simulink model "W08_2_dock"  (R2024b)
settings: Solver=ode4  StartTime=0.0  StopTime=900  FixedStep=Ts_ctrl  RelTol=1e-3
InitFcn:
  | if ~exist('W08_dock_init','file'), addpath(fileparts(get_param('W08_2_dock','FileName'))); end, W08_dock_init('W08_2_dock')
StopFcn:
  | W08_dock_done('W08_2_dock')
values from neighbouring files (symbols this model uses):
  alloc_prm = [half_beam; l_bow; F_max; F_bow_max]    [W08_dock_setup.m]
  animate = 1    [W08_dock_setup.m]    (also in W08_setup.m)
  bow_on = 1    [W08_dock_setup.m]
  Delta = 10    [W08_dock_setup.m]    (also in W08_setup.m)
  dock_q = [dock_north; dock_east; dock_deg*pi/180; L_app; berth_side; R_dock; R_stop]    [W08_dock_setup.m]
  F_bow_max = 250    [W08_dock_setup.m]
  F_max = 500    [W08_dock_setup.m]    (also in W08_setup.m)
  half_beam = 1.027135    [W08_dock_setup.m]    (also in W08_setup.m)
  Izz = 653    [W08_dock_setup.m]    (also in W08_setup.m; build_w08_dock.m = p(2); build_w08_models.m = p(2))
  k_prop = 1000 * 0.004422 * 0.2^4    (= 0.0070752)    [W08_dock_setup.m]    (also in W08_setup.m)
  Kb = Ki_u / Kp_u    (= 0.333333333333)    [W08_dock_setup.m]
  Kd_psi = 200    [W08_dock_setup.m]    (also in W08_setup.m)
  Ki_u = 100    [W08_dock_setup.m]    (also in W08_setup.m)
  Ki_v = 100    [W08_dock_setup.m]
  Kp_psi = 400    [W08_dock_setup.m]    (also in W08_setup.m)
  Kp_u = 300    [W08_dock_setup.m]    (also in W08_setup.m)
  Kp_v = 300    [W08_dock_setup.m]
  Kp_x = 0.4    [W08_dock_setup.m]
  Kp_y = 0.4    [W08_dock_setup.m]
  l_bow = 0.75    [W08_dock_setup.m]
  loiter_radius = 18    [W08_dock_setup.m]    (also in W08_setup.m)
  loiter_turns = 1    [W08_dock_setup.m]    (also in W08_setup.m)
  loiter_wp = 3    [W08_dock_setup.m]    (also in W08_setup.m)
  loiter_xc = wp_north(loiter_wp)    [W08_dock_setup.m]    (also in W08_setup.m)
  loiter_yc = wp_east(loiter_wp)    [W08_dock_setup.m]    (also in W08_setup.m)
  m_usv = 211    [W08_dock_setup.m]    (also in W08_setup.m)
  n_bow_max = sqrt(F_bow_max / k_prop)    [W08_dock_setup.m]
  n_max = sqrt(F_max / k_prop)    [W08_dock_setup.m]    (also in W08_setup.m)
  Nr = 800    [W08_dock_setup.m]    (also in W08_setup.m)
  Nrr = 800    [W08_dock_setup.m]    (also in W08_setup.m; build_w08_dock.m = p(8); build_w08_models.m = p(8))
  p_c = 0.313    [W08_dock_setup.m]    (also in W08_setup.m)
  R_LOS = 5    [W08_dock_setup.m]    (also in W08_setup.m)
  tau_n = 0.30    (= 0.3)    [W08_dock_setup.m]    (also in W08_setup.m)
  Ts_ctrl = 0.05    [W08_dock_setup.m]    (also in W08_setup.m)
  u_max = 1.5    [W08_dock_setup.m]
  u_ref = 1.5    [W08_dock_setup.m]    (also in W08_setup.m)
  v_max = 0.6    [W08_dock_setup.m]
  wp_east = [  20   20   55   90   90 ]    [W08_dock_setup.m]    (also in W08_setup.m)
  wp_north = [ -20   50   20   50   10 ]    [W08_dock_setup.m]    (also in W08_setup.m)
  x0 = [0.1; 0; 0; 0; 0; psi_init]    [W08_dock_setup.m]    (also in W08_setup.m; W08_vrx_run.m = x0old;   x0(6) = psi0;   assignin('base','x0', x0); tidy_layout.m = min(P(:,1)))
  Xu = 100    [W08_dock_setup.m]    (also in W08_setup.m; build_w08_dock.m = p(3); build_w08_models.m = p(3))
  Xuu = 150    [W08_dock_setup.m]    (also in W08_setup.m; build_w08_dock.m = p(4); build_w08_models.m = p(4))
  Yv = 100    [W08_dock_setup.m]    (also in W08_setup.m; build_w08_dock.m = p(5); build_w08_models.m = p(5))
  Yvv = 100    [W08_dock_setup.m]    (also in W08_setup.m; build_w08_dock.m = p(6);'                newline  'Nr=p(7); build_w08_models.m = p(6);'                newline  'Nr=p(7))
libraries: slpidlib x2
settings Model: Creator=admin  LastModifiedBy=admin

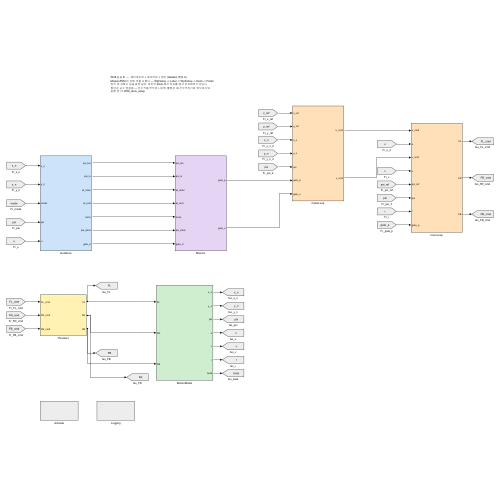
[thumbnail: Simulink's stored preview of the top-level diagram]
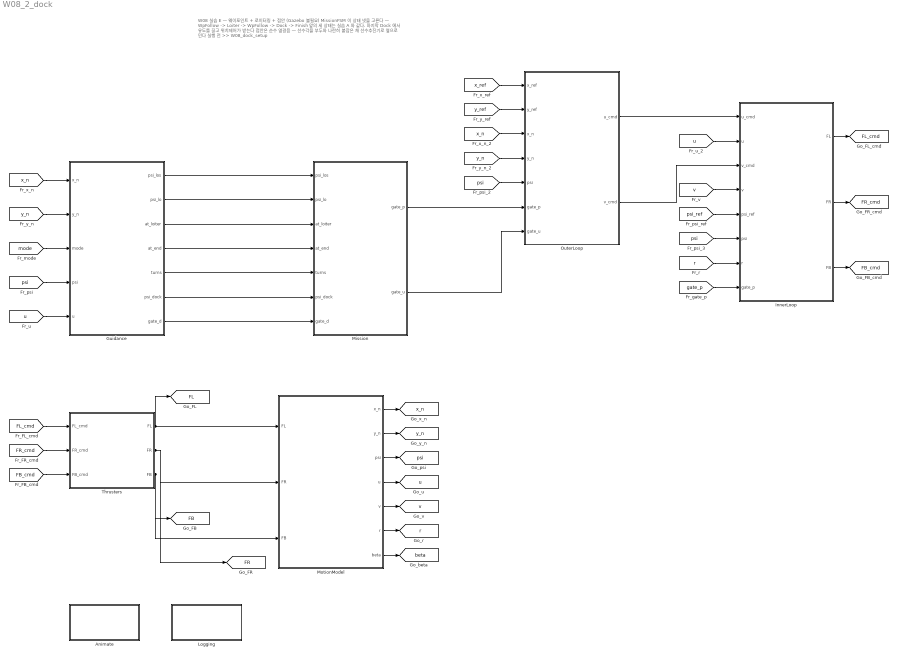
== system W08_2_dock ==
  note: W08 실습 E  —  웨이포인트 + 로이터링 + 접안 (Gazebo 불필요)
      | MissionFSM 이 상태 넷을 고른다 — WpFollow -> Loiter -> WpFollow -> Dock -> Finish
      | 앞의 세 상태는 실습 A 와 같다. 마지막 Dock 에서 유도를 끊고 위치제어가 받는다
      | 접안은 순수 옆걸음 — 선수각을 부두와 나란히 붙잡은 채 선수추진기로 옆으로 민다
      | 실행 전 >> W08_dock_setup
  Animate : Subsystem
  Guidance : Subsystem
  InnerLoop : Subsystem
  Logging : Subsystem
  Mission : Subsystem
  MotionModel : Subsystem
  OuterLoop : Subsystem
  Thrusters : Subsystem
  tag scope: FB=global, FB_cmd=global, FL=global, FL_cmd=global, FR=global, FR_cmd=global, beta=global, psi=global, r=global, u=global, v=global, x_n=global, y_n=global
  wires:
  OuterLoop/2(v_cmd) -> InnerLoop/3(v_cmd)
  OuterLoop/1(u_cmd) -> InnerLoop/1(u_cmd)
  Mission/1(gate_p) -> OuterLoop/6(gate_p)
  Guidance/7(gate_d) -> Mission/7(gate_d)
  Guidance/6(psi_dock) -> Mission/6(psi_dock)
  Guidance/5(turns) -> Mission/5(turns)
  Guidance/4(at_end) -> Mission/4(at_end)
  Guidance/3(at_loiter) -> Mission/3(at_loiter)
  Guidance/2(psi_lo) -> Mission/2(psi_lo)
  Guidance/1(psi_los) -> Mission/1(psi_los)
  Thrusters/2(FR) -> [FR], MotionModel/2(FR)
  Thrusters/1(FL) -> MotionModel/1(FL), [FL]
  Mission/2(gate_u) -> OuterLoop/7(gate_u)
  InnerLoop/1(FL) -> [FL_cmd]
  InnerLoop/2(FR) -> [FR_cmd]
  MotionModel/3(psi) -> [psi]
  MotionModel/4(u) -> [u]
  MotionModel/5(v) -> [v]
  MotionModel/1(x_n) -> [x_n]
  MotionModel/2(y_n) -> [y_n]
  [FL_cmd] -> Thrusters/1(FL_cmd)
  [FR_cmd] -> Thrusters/2(FR_cmd)
  [gate_p] -> InnerLoop/8(gate_p)
  [psi] -> InnerLoop/6(psi)
  [psi_ref] -> InnerLoop/5(psi_ref)
  [r] -> InnerLoop/7(r)
  [u] -> Guidance/5(u)
  [u] -> InnerLoop/2(u)
  [v] -> InnerLoop/4(v)
  [x_ref] -> OuterLoop/1(x_ref)
  [y_ref] -> OuterLoop/2(y_ref)
  InnerLoop/3(FB) -> [FB_cmd]
  MotionModel/7(beta) -> [beta]
  MotionModel/6(r) -> [r]
  [FB_cmd] -> Thrusters/3(FB_cmd)
  [psi] -> Guidance/4(psi)
  [x_n] -> OuterLoop/3(x_n)
  [y_n] -> OuterLoop/4(y_n)
  [mode] -> Guidance/3(mode)
  [psi] -> OuterLoop/5(psi)
  [y_n] -> Guidance/2(y_n)
  [x_n] -> Guidance/1(x_n)
  Thrusters/3(FB) -> [FB], MotionModel/3(FB)

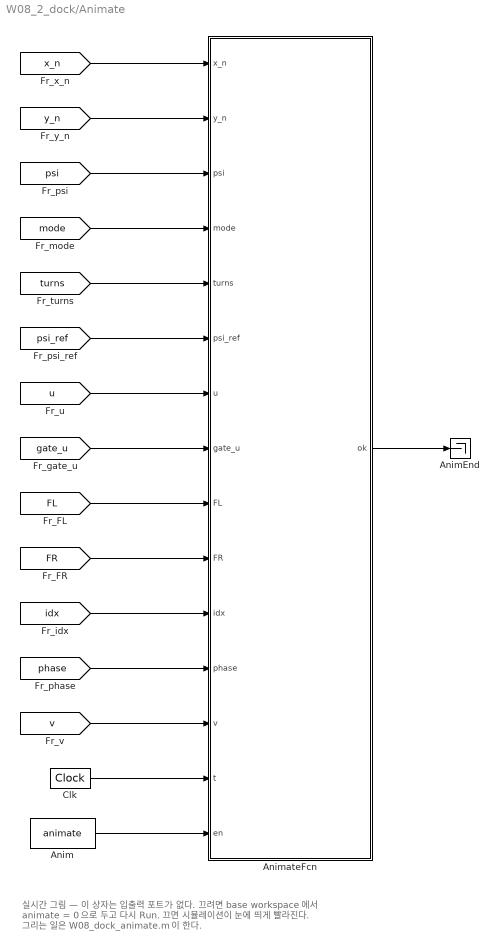
== system W08_2_dock/Animate ==
  note: 실시간 그림 — 이 상자는 입출력 포트가 없다.
      | 끄려면 base workspace 에서  animate = 0  으로 두고 다시 Run.
      | 끄면 시뮬레이션이 눈에 띄게 빨라진다.
      | 그리는 일은 W08_dock_animate.m 이 한다.
  Anim : Constant  Value=animate
  AnimEnd : Terminator
  AnimateFcn : MATLAB Function  TreatAsAtomicUnit=on
  Clk : DigitalClock  SampleTime=Ts_ctrl
  wires:
  [x_n] -> AnimateFcn/1(x_n)
  [y_n] -> AnimateFcn/2(y_n)
  [psi] -> AnimateFcn/3(psi)
  [mode] -> AnimateFcn/4(mode)
  [turns] -> AnimateFcn/5(turns)
  [psi_ref] -> AnimateFcn/6(psi_ref)
  [u] -> AnimateFcn/7(u)
  [gate_u] -> AnimateFcn/8(gate_u)
  [FL] -> AnimateFcn/9(FL)
  [FR] -> AnimateFcn/10(FR)
  [idx] -> AnimateFcn/11(idx)
  [phase] -> AnimateFcn/12(phase)
  [v] -> AnimateFcn/13(v)
  Clk/1 -> AnimateFcn/14(t)
  Anim/1 -> AnimateFcn/15(en)
  AnimateFcn/1(ok) -> AnimEnd/1

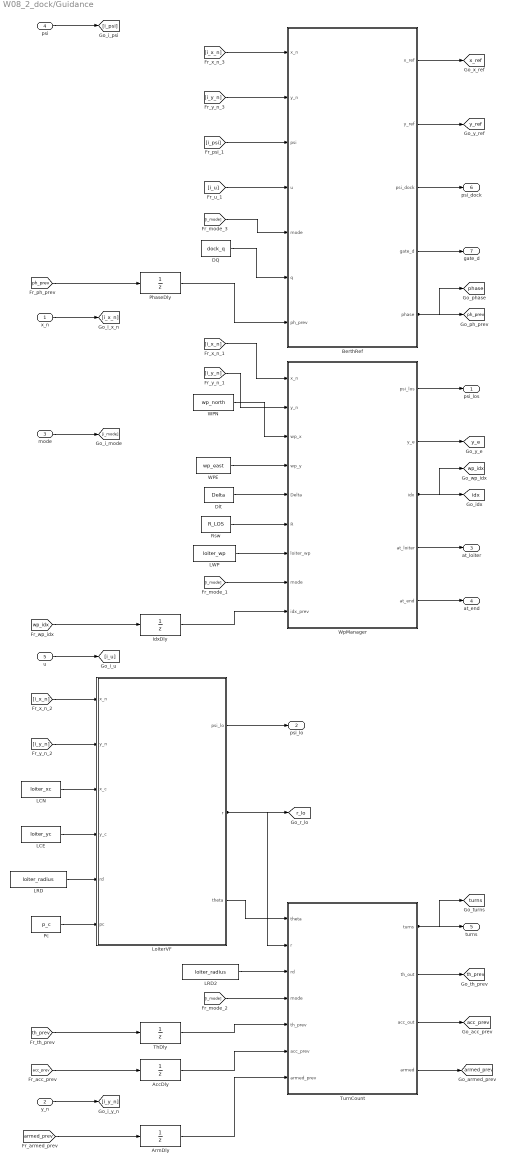
== system W08_2_dock/Guidance ==
  x_n : Inport
  y_n : Inport  Port=2
  mode : Inport  Port=3
  psi : Inport  Port=4
  u : Inport  Port=5
  AccDly : UnitDelay  Description=바퀴 수 계수기 — 표본 사이의 각 변화를 모아 감으므로 바로 앞 표본이 있어야 한다. 또한 TurnCount 가 낸 값이 TurnCount 로 되돌아와 대수 루프가 된다.  SampleTime=Ts_ctrl  HasFrameUpgradeWarning=on
  ArmDly : UnitDelay  Description=바퀴 수 계수기 — 표본 사이의 각 변화를 모아 감으므로 바로 앞 표본이 있어야 한다. 또한 TurnCount 가 낸 값이 TurnCount 로 되돌아와 대수 루프가 된다.  SampleTime=Ts_ctrl  HasFrameUpgradeWarning=on
  BerthRef : MATLAB Function  TreatAsAtomicUnit=on
  DQ : Constant  Value=dock_q
  Dlt : Constant  Value=Delta
  IdxDly : UnitDelay  Description=대수 루프 차단 + 사건 계수기 — 웨이포인트 번호는 정수이고, 유도부가 낸 값이 유도부로 되돌아온다. 미분방정식의 상태가 아니다.  InitialCondition=1  SampleTime=Ts_ctrl  HasFrameUpgradeWarning=on
  LCE : Constant  Value=loiter_yc
  LCN : Constant  Value=loiter_xc
  LRD : Constant  Value=loiter_radius
  LRD2 : Constant  Value=loiter_radius
  LWP : Constant  Value=loiter_wp
  LoiterVF : MATLAB Function  TreatAsAtomicUnit=on
  Pc : Constant  Value=p_c
  PhaseDly : UnitDelay  Description=대수 루프 차단 + 단계 걸쇠 — 접안 단계는 정수이고, 한 번 올라간 단계는 내려오지 않는다. 미분방정식의 상태가 아니다.  SampleTime=Ts_ctrl  HasFrameUpgradeWarning=on
  Rsw : Constant  Value=R_LOS
  ThDly : UnitDelay  Description=바퀴 수 계수기 — 표본 사이의 각 변화를 모아 감으므로 바로 앞 표본이 있어야 한다. 또한 TurnCount 가 낸 값이 TurnCount 로 되돌아와 대수 루프가 된다.  SampleTime=Ts_ctrl  HasFrameUpgradeWarning=on
  TurnCount : MATLAB Function  TreatAsAtomicUnit=on
  WPE : Constant  Value=wp_east
  WPN : Constant  Value=wp_north
  WpManager : MATLAB Function  TreatAsAtomicUnit=on
  psi_los : Outport
  psi_lo : Outport  Port=2
  at_loiter : Outport  Port=3
  at_end : Outport  Port=4
  turns : Outport  Port=5
  psi_dock : Outport  Port=6
  gate_d : Outport  Port=7
  tag scope: acc_prev=global, armed_prev=global, idx=global, ph_prev=global, phase=global, r_lo=global, th_prev=global, turns=global, wp_idx=global, x_ref=global, y_e=global, y_ref=global
  wires:
  WpManager/4(at_loiter) -> at_loiter/1
  psi/1 -> [i_psi]
  mode/1 -> [i_mode]
  LCE/1 -> LoiterVF/4(y_c)
  [ph_prev] -> PhaseDly/1
  LRD/1 -> LoiterVF/5(rd)
  x_n/1 -> [i_x_n]
  WpManager/5(at_end) -> at_end/1
  [wp_idx] -> IdxDly/1
  TurnCount/1(turns) -> turns/1, [turns]
  u/1 -> [i_u]
  [i_x_n] -> LoiterVF/1(x_n)
  WPE/1 -> WpManager/4(wp_y)
  [i_y_n] -> WpManager/2(y_n)
  [i_y_n] -> LoiterVF/2(y_n)
  WpManager/3(idx) -> [wp_idx], [idx]
  LCN/1 -> LoiterVF/3(x_c)
  Pc/1 -> LoiterVF/6(pc)
  [th_prev] -> ThDly/1
  [acc_prev] -> AccDly/1
  y_n/1 -> [i_y_n]
  [armed_prev] -> ArmDly/1
  [i_x_n] -> BerthRef/1(x_n)
  [i_y_n] -> BerthRef/2(y_n)
  [i_psi] -> BerthRef/3(psi)
  [i_u] -> BerthRef/4(u)
  [i_mode] -> BerthRef/5(mode)
  DQ/1 -> BerthRef/6(q)
  PhaseDly/1 -> BerthRef/7(ph_prev)
  [i_x_n] -> WpManager/1(x_n)
  WPN/1 -> WpManager/3(wp_x)
  Dlt/1 -> WpManager/5(Delta)
  Rsw/1 -> WpManager/6(R)
  LWP/1 -> WpManager/7(loiter_wp)
  BerthRef/4(gate_d) -> gate_d/1
  [i_mode] -> WpManager/8(mode)
  IdxDly/1 -> WpManager/9(idx_prev)
  LoiterVF/1(psi_lo) -> psi_lo/1
  LoiterVF/2(r) -> [r_lo], TurnCount/2(r)
  LoiterVF/3(theta) -> TurnCount/1(theta)
  LRD2/1 -> TurnCount/3(rd)
  [i_mode] -> TurnCount/4(mode)
  TurnCount/3(acc_out) -> [acc_prev]
  BerthRef/2(y_ref) -> [y_ref]
  ThDly/1 -> TurnCount/5(th_prev)
  AccDly/1 -> TurnCount/6(acc_prev)
  WpManager/2(y_e) -> [y_e]
  ArmDly/1 -> TurnCount/7(armed_prev)
  BerthRef/5(phase) -> [ph_prev], [phase]
  BerthRef/1(x_ref) -> [x_ref]
  BerthRef/3(psi_dock) -> psi_dock/1
  WpManager/1(psi_los) -> psi_los/1
  TurnCount/2(th_out) -> [th_prev]
  TurnCount/4(armed) -> [armed_prev]

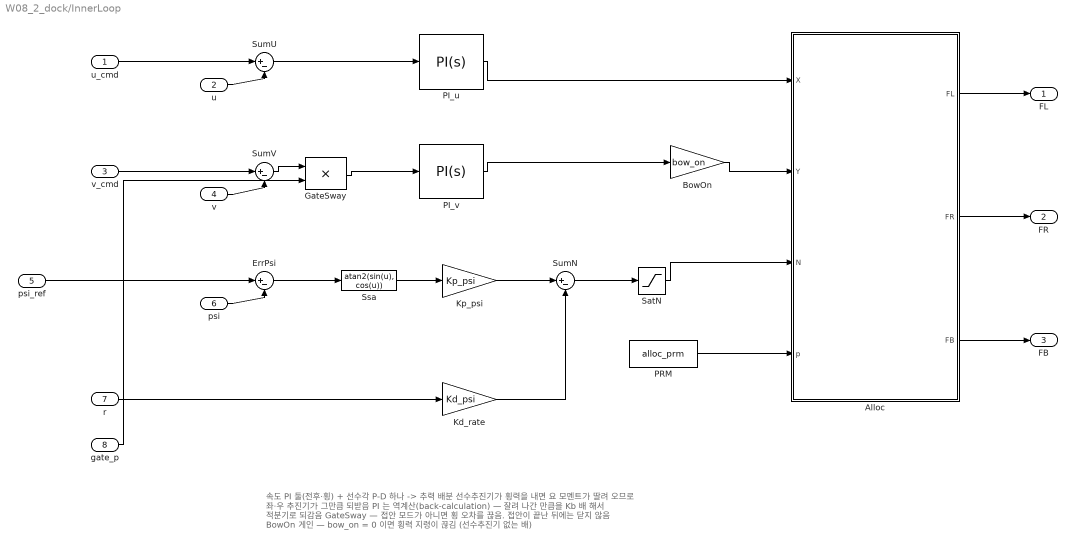
== system W08_2_dock/InnerLoop ==
  note: 속도 PI 둘(전후·횡) + 선수각 P-D 하나 -> 추력 배분
      | 선수추진기가 횡력을 내면 요 모멘트가 딸려 오므로 좌·우 추진기가 그만큼 되받음
      | PI 는 역계산(back-calculation) — 잘려 나간 만큼을 Kb 배 해서 적분기로 되감음
      | GateSway — 접안 모드가 아니면 횡 오차를 끊음. 접안이 끝난 뒤에는 닫지 않음
      | BowOn 게인 — bow_on = 0 이면 횡력 지령이 끊김 (선수추진기 없는 배)
  u_cmd : Inport
  u : Inport  Port=2
  v_cmd : Inport  Port=3
  v : Inport  Port=4
  psi_ref : Inport  Port=5
  psi : Inport  Port=6
  r : Inport  Port=7
  gate_p : Inport  Port=8
  Alloc : MATLAB Function  TreatAsAtomicUnit=on
  BowOn : Gain  Gain=bow_on
  ErrPsi : Sum  Inputs=|+-
  GateSway : Product
  Kd_rate : Gain  Gain=Kd_psi
  Kp_psi : Gain  Gain=Kp_psi
  PI_u : slpidlib/PID Controller  Controller=PI  Form=Parallel  TimeDomain=Continuous-time  UseExternalTs=off  SampleTime=-1  IntegratorMethod=Forward Euler  FilterMethod=Forward Euler  ControllerParametersSource=internal  P=Kp_u  I=Ki_u  UseKiTs=off  D=0  UseExternalDerivativeSource=off  N=100  UseFilter=on  TunerSelectOption=Transfer Function Based (PID Tuner App)  InitialConditionSource=internal  InitialConditionForIntegrator=0  InitialConditionForFilter=0  DifferentiatorICPrevScaledInput=0  ExternalReset=none  TrackingMode=off  Kt=1  LimitOutput=on  SatLimitsSource=internal  UpperSaturationLimit=2*F_max  LowerSaturationLimit=-(2*F_max)  LinearizeAsGain=on  AntiWindupMode=back-calculation  Kb=Kb  LimitIntegrator=off  UpperIntegratorSaturationLimit=inf  LowerIntegratorSaturationLimit=-inf  POutMin=[]  POutMax=[]  IOutMin=[]  IOutMax=[]  DOutMin=[]  DOutMax=[]  NOutMin=[]  NOutMax=[]  SumOutMin=[]  SumOutMax=[]  SaturationOutMin=[]  SaturationOutMax=[]  PParamMin=[]  PParamMax=[]  IParamMin=[]  IParamMax=[]  DParamMin=[]  DParamMax=[]  NParamMin=[]  NParamMax=[]  KbParamMin=[]  KbParamMax=[]  KtParamMin=[]  KtParamMax=[]  KbOutMin=[]  KbOutMax=[]  KtOutMin=[]  KtOutMax=[]  IntegratorOutMin=[]  IntegratorOutMax=[]  FilterOutMin=[]  FilterOutMax=[]  SumI1OutMin=[]  SumI1OutMax=[]  SumI2OutMin=[]  SumI2OutMax=[]  SumI3OutMin=[]  SumI3OutMax=[]  SumI4OutMin=[]  SumI4OutMax=[]  SumDOutMin=[]  SumDOutMax=[]  DifferentiatorOutMin=[]  DifferentiatorOutMax=[]  FilterDiffOutCoefMin=[]  FilterDiffOutCoefMax=[]  ReciprocalOutMin=[]  ReciprocalOutMax=[]  SumDenOutMin=[]  SumDenOutMax=[]  SumNumOutMin=[]  SumNumOutMax=[]  DivideOutMin=[]  DivideOutMax=[]  UdiffTsProdOutMin=[]  UdiffTsProdOutMax=[]  NTsProdOutMin=[]  NTsProdOutMax=[]  UintegralTsProdOutMin=[]  UintegralTsProdOutMax=[]  UngainTsProdOutMin=[]  UngainTsProdOutMax=[]  ClampingZeroOutDataTypeStr=Inherit: Inherit via back propagation  ClampingZeroOutMin=[]  ClampingZeroOutMax=[]  FilterDenConstantOutDataTypeStr=Inherit: Inherit via back propagation  FilterDenConstantOutMin=[]  FilterDenConstantOutMax=[]  PCopyOutDataTypeStr=Inherit: Inherit via back propagation  PCopyOutMin=[]  PCopyOutMax=[]  NCopyOutDataTypeStr=Inherit: Inherit via back propagation  NCopyOutMin=[]  NCopyOutMax=[]  IntegratorContinuousStateAttributes=''  IntegratorStateMustResolveToSignalObject=off  IntegratorRTWStateStorageClass=Auto  FilterContinuousStateAttributes=''  FilterStateMustResolveToSignalObject=off  FilterRTWStateStorageClass=Auto  ParallelPVariant=InternalParameters  IdealPVariant=Disabled  IVariant=InternalParameters  DVariant=Disabled  IntegratorVariant=Continuous  SatVariant=Enabled  AWVariant=BackCalculation  PCopyVariant=Disabled  TRVariant=Disabled  FdbkBlocksVariant=Forward  IdealPFdbkVariant=Disabled  SatFdbkVariant=Disabled  DerivativeFilterVariant=Disabled  NVariant=Disabled  NCopyVariant=Disabled_SignalSpec  FilterICVariant=Disabled  IntegratorICVariant=InternalICs  ExternalResetVariant=Disabled  TRSumVariant=Passthrough  SumFdbkVariant=Disabled  SumVariant=Sum_PI  TsampFilterVariant=InternalTs  TsampNgainVariant=Passthrough  TsampIntegralVariant=Disabled_SignalSpec  ExternalSaturationOutDataTypeStr=Inherit: Same as second input  DerivativeSourceVariant=Disabled  PreIntVariant=InternalPreInt
  PI_v : slpidlib/PID Controller  Controller=PI  Form=Parallel  TimeDomain=Continuous-time  UseExternalTs=off  SampleTime=-1  IntegratorMethod=Forward Euler  FilterMethod=Forward Euler  ControllerParametersSource=internal  P=Kp_v  I=Ki_v  UseKiTs=off  D=0  UseExternalDerivativeSource=off  N=100  UseFilter=on  TunerSelectOption=Transfer Function Based (PID Tuner App)  InitialConditionSource=internal  InitialConditionForIntegrator=0  InitialConditionForFilter=0  DifferentiatorICPrevScaledInput=0  ExternalReset=none  TrackingMode=off  Kt=1  LimitOutput=on  SatLimitsSource=internal  UpperSaturationLimit=F_bow_max  LowerSaturationLimit=-(F_bow_max)  LinearizeAsGain=on  AntiWindupMode=back-calculation  Kb=Kb  LimitIntegrator=off  UpperIntegratorSaturationLimit=inf  LowerIntegratorSaturationLimit=-inf  POutMin=[]  POutMax=[]  IOutMin=[]  IOutMax=[]  DOutMin=[]  DOutMax=[]  NOutMin=[]  NOutMax=[]  SumOutMin=[]  SumOutMax=[]  SaturationOutMin=[]  SaturationOutMax=[]  PParamMin=[]  PParamMax=[]  IParamMin=[]  IParamMax=[]  DParamMin=[]  DParamMax=[]  NParamMin=[]  NParamMax=[]  KbParamMin=[]  KbParamMax=[]  KtParamMin=[]  KtParamMax=[]  KbOutMin=[]  KbOutMax=[]  KtOutMin=[]  KtOutMax=[]  IntegratorOutMin=[]  IntegratorOutMax=[]  FilterOutMin=[]  FilterOutMax=[]  SumI1OutMin=[]  SumI1OutMax=[]  SumI2OutMin=[]  SumI2OutMax=[]  SumI3OutMin=[]  SumI3OutMax=[]  SumI4OutMin=[]  SumI4OutMax=[]  SumDOutMin=[]  SumDOutMax=[]  DifferentiatorOutMin=[]  DifferentiatorOutMax=[]  FilterDiffOutCoefMin=[]  FilterDiffOutCoefMax=[]  ReciprocalOutMin=[]  ReciprocalOutMax=[]  SumDenOutMin=[]  SumDenOutMax=[]  SumNumOutMin=[]  SumNumOutMax=[]  DivideOutMin=[]  DivideOutMax=[]  UdiffTsProdOutMin=[]  UdiffTsProdOutMax=[]  NTsProdOutMin=[]  NTsProdOutMax=[]  UintegralTsProdOutMin=[]  UintegralTsProdOutMax=[]  UngainTsProdOutMin=[]  UngainTsProdOutMax=[]  ClampingZeroOutDataTypeStr=Inherit: Inherit via back propagation  ClampingZeroOutMin=[]  ClampingZeroOutMax=[]  FilterDenConstantOutDataTypeStr=Inherit: Inherit via back propagation  FilterDenConstantOutMin=[]  FilterDenConstantOutMax=[]  PCopyOutDataTypeStr=Inherit: Inherit via back propagation  PCopyOutMin=[]  PCopyOutMax=[]  NCopyOutDataTypeStr=Inherit: Inherit via back propagation  NCopyOutMin=[]  NCopyOutMax=[]  IntegratorContinuousStateAttributes=''  IntegratorStateMustResolveToSignalObject=off  IntegratorRTWStateStorageClass=Auto  FilterContinuousStateAttributes=''  FilterStateMustResolveToSignalObject=off  FilterRTWStateStorageClass=Auto  ParallelPVariant=InternalParameters  IdealPVariant=Disabled  IVariant=InternalParameters  DVariant=Disabled  IntegratorVariant=Continuous  SatVariant=Enabled  AWVariant=BackCalculation  PCopyVariant=Disabled  TRVariant=Disabled  FdbkBlocksVariant=Forward  IdealPFdbkVariant=Disabled  SatFdbkVariant=Disabled  DerivativeFilterVariant=Disabled  NVariant=Disabled  NCopyVariant=Disabled_SignalSpec  FilterICVariant=Disabled  IntegratorICVariant=InternalICs  ExternalResetVariant=Disabled  TRSumVariant=Passthrough  SumFdbkVariant=Disabled  SumVariant=Sum_PI  TsampFilterVariant=InternalTs  TsampNgainVariant=Passthrough  TsampIntegralVariant=Disabled_SignalSpec  ExternalSaturationOutDataTypeStr=Inherit: Same as second input  DerivativeSourceVariant=Disabled  PreIntVariant=InternalPreInt
  PRM : Constant  Value=alloc_prm
  SatN : Saturate  UpperLimit=2*F_max*half_beam + F_bow_max*l_bow  LowerLimit=-(2*F_max*half_beam + F_bow_max*l_bow)
  Ssa : Fcn  Expr=atan2(sin(u), cos(u))
  SumN : Sum  Inputs=|+-
  SumU : Sum  Inputs=|+-
  SumV : Sum  Inputs=|+-
  FL : Outport
  FR : Outport  Port=2
  FB : Outport  Port=3
  wires:
  u_cmd/1 -> SumU/1
  u/1 -> SumU/2
  v_cmd/1 -> SumV/1
  v/1 -> SumV/2
  SumV/1 -> GateSway/1
  gate_p/1 -> GateSway/2
  SumU/1 -> PI_u/1
  GateSway/1 -> PI_v/1
  ErrPsi/1 -> Ssa/1
  psi_ref/1 -> ErrPsi/1
  psi/1 -> ErrPsi/2
  Ssa/1 -> Kp_psi/1
  r/1 -> Kd_rate/1
  Kp_psi/1 -> SumN/1
  Kd_rate/1 -> SumN/2
  SumN/1 -> SatN/1
  PI_u/1 -> Alloc/1(X)
  PI_v/1 -> BowOn/1
  BowOn/1 -> Alloc/2(Y)
  SatN/1 -> Alloc/3(N)
  PRM/1 -> Alloc/4(p)
  Alloc/1(FL) -> FL/1
  Alloc/2(FR) -> FR/1
  Alloc/3(FB) -> FB/1

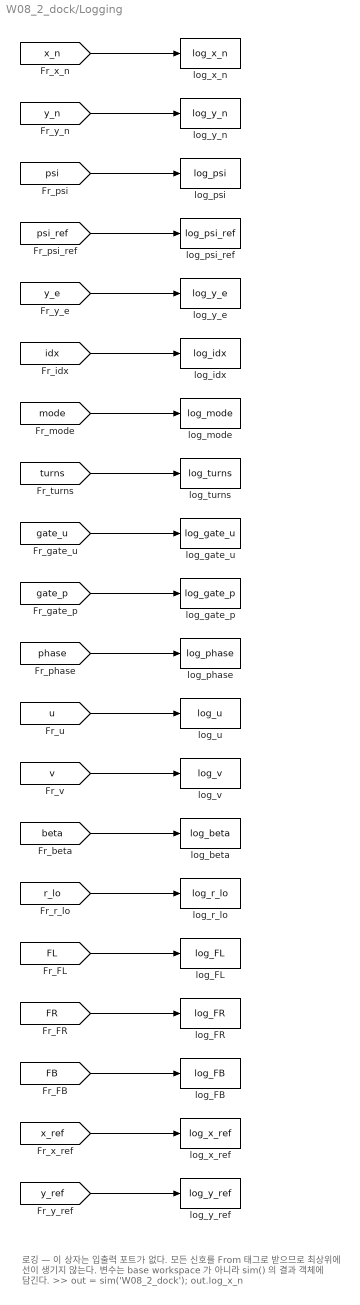
== system W08_2_dock/Logging ==
  note: 로깅 — 이 상자는 입출력 포트가 없다.
      | 모든 신호를 From 태그로 받으므로 최상위에 선이 생기지 않는다.
      | 변수는 base workspace 가 아니라 sim() 의 결과 객체에 담긴다.
      |   >> out = sim('W08_2_dock');  out.log_x_n
  log_FB : ToWorkspace  VariableName=log_FB  SaveFormat=Timeseries  SampleTime=Ts_ctrl
  log_FL : ToWorkspace  VariableName=log_FL  SaveFormat=Timeseries  SampleTime=Ts_ctrl
  log_FR : ToWorkspace  VariableName=log_FR  SaveFormat=Timeseries  SampleTime=Ts_ctrl
  log_beta : ToWorkspace  VariableName=log_beta  SaveFormat=Timeseries  SampleTime=Ts_ctrl
  log_gate_p : ToWorkspace  VariableName=log_gate_p  SaveFormat=Timeseries  SampleTime=Ts_ctrl
  log_gate_u : ToWorkspace  VariableName=log_gate_u  SaveFormat=Timeseries  SampleTime=Ts_ctrl
  log_idx : ToWorkspace  VariableName=log_idx  SaveFormat=Timeseries  SampleTime=Ts_ctrl
  log_mode : ToWorkspace  VariableName=log_mode  SaveFormat=Timeseries  SampleTime=Ts_ctrl
  log_phase : ToWorkspace  VariableName=log_phase  SaveFormat=Timeseries  SampleTime=Ts_ctrl
  log_psi : ToWorkspace  VariableName=log_psi  SaveFormat=Timeseries  SampleTime=Ts_ctrl
  log_psi_ref : ToWorkspace  VariableName=log_psi_ref  SaveFormat=Timeseries  SampleTime=Ts_ctrl
  log_r_lo : ToWorkspace  VariableName=log_r_lo  SaveFormat=Timeseries  SampleTime=Ts_ctrl
  log_turns : ToWorkspace  VariableName=log_turns  SaveFormat=Timeseries  SampleTime=Ts_ctrl
  log_u : ToWorkspace  VariableName=log_u  SaveFormat=Timeseries  SampleTime=Ts_ctrl
  log_v : ToWorkspace  VariableName=log_v  SaveFormat=Timeseries  SampleTime=Ts_ctrl
  log_x_n : ToWorkspace  VariableName=log_x_n  SaveFormat=Timeseries  SampleTime=Ts_ctrl
  log_x_ref : ToWorkspace  VariableName=log_x_ref  SaveFormat=Timeseries  SampleTime=Ts_ctrl
  log_y_e : ToWorkspace  VariableName=log_y_e  SaveFormat=Timeseries  SampleTime=Ts_ctrl
  log_y_n : ToWorkspace  VariableName=log_y_n  SaveFormat=Timeseries  SampleTime=Ts_ctrl
  log_y_ref : ToWorkspace  VariableName=log_y_ref  SaveFormat=Timeseries  SampleTime=Ts_ctrl
  wires:
  [x_n] -> log_x_n/1
  [y_n] -> log_y_n/1
  [psi] -> log_psi/1
  [psi_ref] -> log_psi_ref/1
  [y_e] -> log_y_e/1
  [idx] -> log_idx/1
  [mode] -> log_mode/1
  [turns] -> log_turns/1
  [gate_u] -> log_gate_u/1
  [gate_p] -> log_gate_p/1
  [phase] -> log_phase/1
  [u] -> log_u/1
  [v] -> log_v/1
  [beta] -> log_beta/1
  [r_lo] -> log_r_lo/1
  [FL] -> log_FL/1
  [FR] -> log_FR/1
  [FB] -> log_FB/1
  [x_ref] -> log_x_ref/1
  [y_ref] -> log_y_ref/1

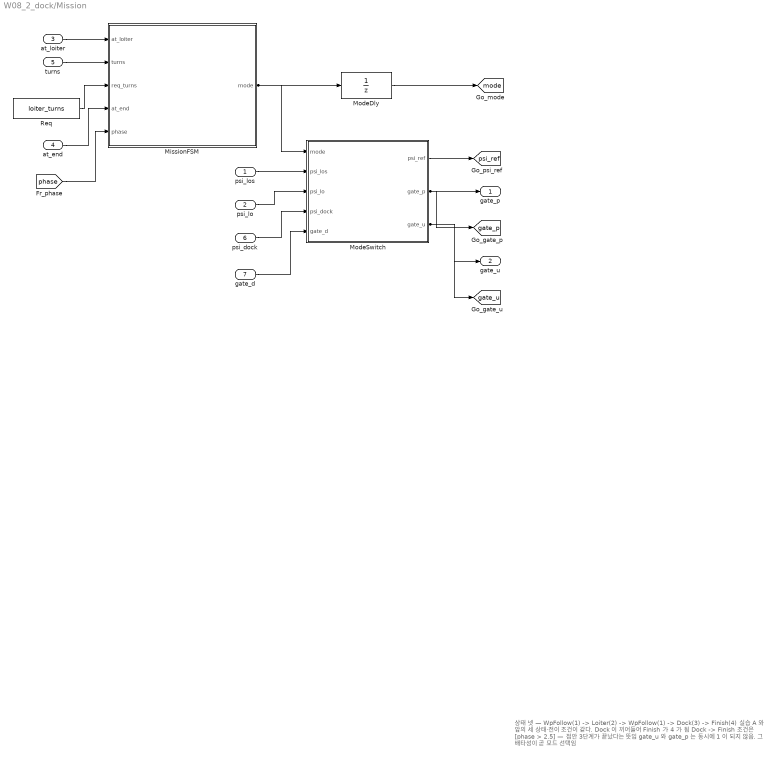
== system W08_2_dock/Mission ==
  note: 상태 넷 — WpFollow(1) -> Loiter(2) -> WpFollow(1) -> Dock(3) -> Finish(4)
      | 실습 A 와 앞의 세 상태·전이 조건이 같다. Dock 이 끼어들어 Finish 가 4 가 됨
      | Dock -> Finish 조건은 [phase > 2.5] — 접안 3단계가 끝났다는 뜻임
      | gate_u 와 gate_p 는 동시에 1 이 되지 않음. 그 배타성이 곧 모드 선택임
  psi_los : Inport
  psi_lo : Inport  Port=2
  at_loiter : Inport  Port=3
  at_end : Inport  Port=4
  turns : Inport  Port=5
  psi_dock : Inport  Port=6
  gate_d : Inport  Port=7
  MissionFSM : Stateflow chart  TreatAsAtomicUnit=on
  ModeDly : UnitDelay  Description=대수 루프 차단 — 상태기계가 낸 mode 가 유도부로 돌아가고, 유도부가 낸 at_loiter·at_end·turns·phase 가 다시 상태기계로 들어온다. 고리 어딘가에 한 스텝 지연이 있어야 한다.  InitialCondition=1  SampleTime=Ts_ctrl  HasFrameUpgradeWarning=on
  ModeSwitch : MATLAB Function  TreatAsAtomicUnit=on
  Req : Constant  Value=loiter_turns
  gate_p : Outport
  gate_u : Outport  Port=2
  tag scope: gate_p=global, gate_u=global, mode=global, psi_ref=global
  wires:
  psi_lo/1 -> ModeSwitch/3(psi_lo)
  at_loiter/1 -> MissionFSM/1(at_loiter)
  psi_los/1 -> ModeSwitch/2(psi_los)
  Req/1 -> MissionFSM/3(req_turns)
  turns/1 -> MissionFSM/2(turns)
  at_end/1 -> MissionFSM/4(at_end)
  MissionFSM/1(mode) -> ModeSwitch/1(mode), ModeDly/1
  [phase] -> MissionFSM/5(phase)
  psi_dock/1 -> ModeSwitch/4(psi_dock)
  gate_d/1 -> ModeSwitch/5(gate_d)
  ModeDly/1 -> [mode]
  ModeSwitch/3(gate_u) -> gate_u/1, [gate_u]
  ModeSwitch/1(psi_ref) -> [psi_ref]
  ModeSwitch/2(gate_p) -> [gate_p], gate_p/1

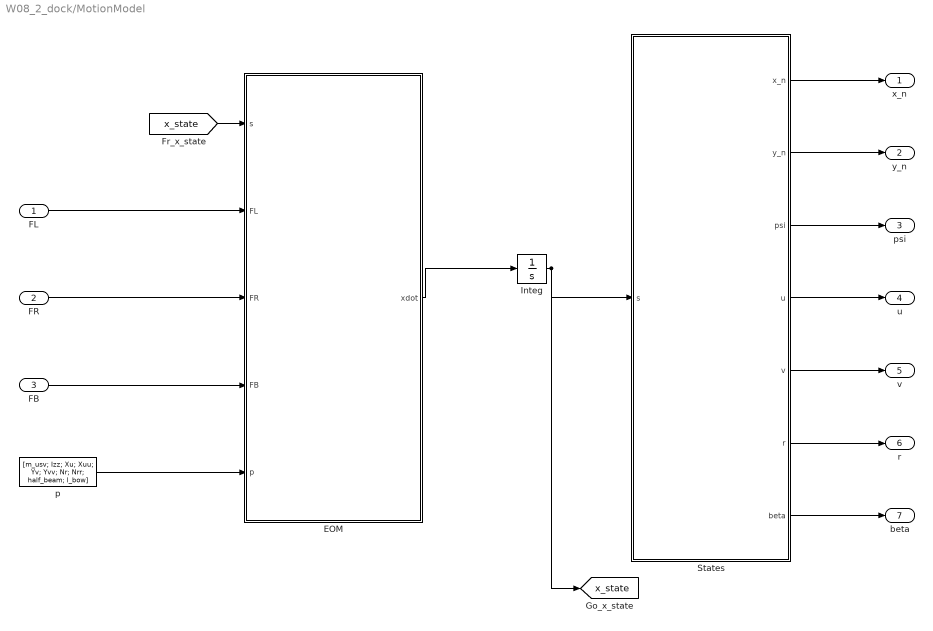
== system W08_2_dock/MotionModel ==
  FL : Inport
  FR : Inport  Port=2
  FB : Inport  Port=3
  EOM : MATLAB Function  TreatAsAtomicUnit=on
  Integ : Integrator  InitialCondition=x0
  States : MATLAB Function  TreatAsAtomicUnit=on
  p : Constant  Value=[m_usv; Izz; Xu; Xuu; Yv; Yvv; Nr; Nrr; half_beam; l_bow]
  x_n : Outport
  y_n : Outport  Port=2
  psi : Outport  Port=3
  u : Outport  Port=4
  v : Outport  Port=5
  r : Outport  Port=6
  beta : Outport  Port=7
  tag scope: x_state=global
  wires:
  FL/1 -> EOM/2(FL)
  FR/1 -> EOM/3(FR)
  FB/1 -> EOM/4(FB)
  p/1 -> EOM/5(p)
  EOM/1(xdot) -> Integ/1
  Integ/1 -> States/1(s), [x_state]
  [x_state] -> EOM/1(s)
  States/1(x_n) -> x_n/1
  States/2(y_n) -> y_n/1
  States/3(psi) -> psi/1
  States/4(u) -> u/1
  States/5(v) -> v/1
  States/6(r) -> r/1
  States/7(beta) -> beta/1

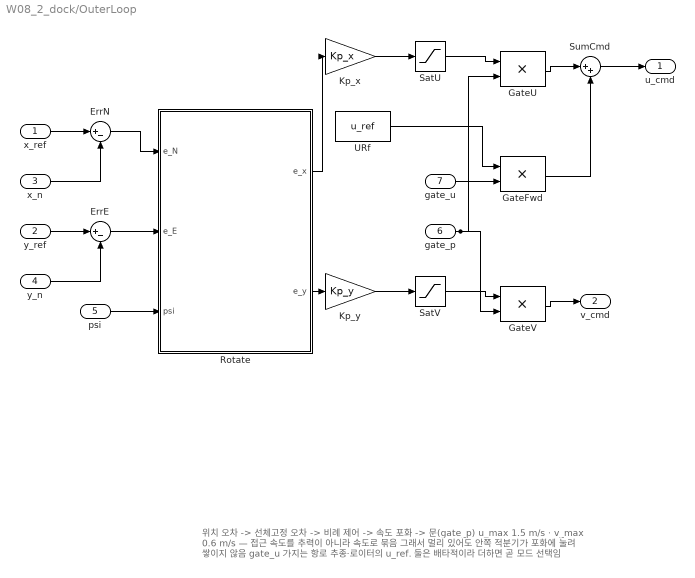
== system W08_2_dock/OuterLoop ==
  note: 위치 오차 -> 선체고정 오차 -> 비례 제어 -> 속도 포화 -> 문(gate_p)
      | u_max 1.5 m/s · v_max 0.6 m/s — 접근 속도를 추력이 아니라 속도로 묶음
      | 그래서 멀리 있어도 안쪽 적분기가 포화에 눌려 쌓이지 않음
      | gate_u 가지는 항로 추종·로이터의 u_ref. 둘은 배타적이라 더하면 곧 모드 선택임
  x_ref : Inport
  y_ref : Inport  Port=2
  x_n : Inport  Port=3
  y_n : Inport  Port=4
  psi : Inport  Port=5
  gate_p : Inport  Port=6
  gate_u : Inport  Port=7
  ErrE : Sum  Inputs=|+-
  ErrN : Sum  Inputs=|+-
  GateFwd : Product
  GateU : Product
  GateV : Product
  Kp_x : Gain  Gain=Kp_x
  Kp_y : Gain  Gain=Kp_y
  Rotate : MATLAB Function  TreatAsAtomicUnit=on
  SatU : Saturate  UpperLimit=u_max  LowerLimit=-(u_max)
  SatV : Saturate  UpperLimit=v_max  LowerLimit=-(v_max)
  SumCmd : Sum  Inputs=|++
  URf : Constant  Value=u_ref
  u_cmd : Outport
  v_cmd : Outport  Port=2
  wires:
  y_n/1 -> ErrE/2
  ErrN/1 -> Rotate/1(e_N)
  x_ref/1 -> ErrN/1
  SatU/1 -> GateU/1
  x_n/1 -> ErrN/2
  psi/1 -> Rotate/3(psi)
  y_ref/1 -> ErrE/1
  Rotate/1(e_x) -> Kp_x/1
  ErrE/1 -> Rotate/2(e_E)
  Rotate/2(e_y) -> Kp_y/1
  gate_p/1 -> GateU/2, GateV/2
  Kp_x/1 -> SatU/1
  Kp_y/1 -> SatV/1
  URf/1 -> GateFwd/1
  gate_u/1 -> GateFwd/2
  SatV/1 -> GateV/1
  SumCmd/1 -> u_cmd/1
  GateU/1 -> SumCmd/1
  GateFwd/1 -> SumCmd/2
  GateV/1 -> v_cmd/1

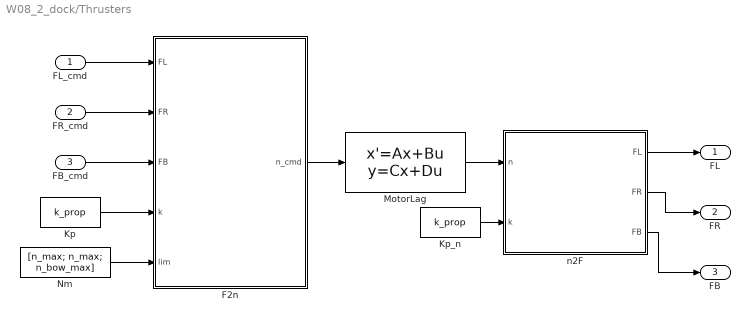
== system W08_2_dock/Thrusters ==
  FL_cmd : Inport
  FR_cmd : Inport  Port=2
  FB_cmd : Inport  Port=3
  F2n : MATLAB Function  TreatAsAtomicUnit=on
  Kp : Constant  Value=k_prop
  Kp_n : Constant  Value=k_prop
  MotorLag : StateSpace  A=-eye(3)/tau_n  B=eye(3)/tau_n  C=eye(3)  D=zeros(3)  InitialCondition=zeros(3,1)
  Nm : Constant  Value=[n_max; n_max; n_bow_max]
  n2F : MATLAB Function  TreatAsAtomicUnit=on
  FL : Outport
  FR : Outport  Port=2
  FB : Outport  Port=3
  wires:
  FL_cmd/1 -> F2n/1(FL)
  Nm/1 -> F2n/5(lim)
  FR_cmd/1 -> F2n/2(FR)
  F2n/1(n_cmd) -> MotorLag/1
  FB_cmd/1 -> F2n/3(FB)
  Kp/1 -> F2n/4(k)
  MotorLag/1 -> n2F/1(n)
  Kp_n/1 -> n2F/2(k)
  n2F/1(FL) -> FL/1
  n2F/2(FR) -> FR/1
  n2F/3(FB) -> FB/1

== matlab function W08_2_dock/Mission/ModeSwitch ==
  data: mode input; psi_ref output; psi_los input; psi_lo input; psi_dock input; gate_d input; gate_p output; gate_u output
function [psi_ref, gate_p, gate_u] = ModeSwitch(mode, psi_los, psi_lo, psi_dock, gate_d)
%#codegen
%  상태 번호를 받아 **쓸 지령**을 고른다. 판단은 상태기계가 이미 끝냈다.
%
%    mode 1 WpFollow   LOS 선수각,        전진 속도 u_ref
%    mode 2 Loiter     벡터필드 선수각,   전진 속도 u_ref
%    mode 3 Dock       부두 선수각,       전진·횡 속도는 위치제어가 낸다
%    mode 4 Finish     부두 선수각,       위치제어로 선석을 지킨다
%
%  선수각 고리는 어느 모드에서도 **끊지 않는다.** Finish 에서도 선수각은
%  부두와 나란히 붙잡아야 접안 자세가 풀리지 않는다
if mode > 3.5
    psi_ref = psi_dock;   gate_p = gate_d;   gate_u = 0;
elseif mode > 2.5
    psi_ref = psi_dock;   gate_p = gate_d;   gate_u = 0;
elseif mode > 1.5
    psi_ref = psi_lo;     gate_p = 0;        gate_u = 1;
else
    psi_ref = psi_los;    gate_p = 0;        gate_u = 1;
end

== matlab function W08_2_dock/OuterLoop/Rotate ==
  data: e_N input; e_x output; e_E input; psi input; e_y output
function [e_x, e_y] = Rotate(e_N, e_E, psi)
%#codegen
%  NED 위치 오차를 선체고정 오차로 돌린다. e_x 앞쪽, e_y 우현쪽 [m]
e_x =  cos(psi)*e_N + sin(psi)*e_E;
e_y = -sin(psi)*e_N + cos(psi)*e_E;

== matlab function W08_2_dock/InnerLoop/Alloc ==
  data: X input; FL output; Y input; N input; p input; FR output; FB output
function [FL, FR, FB] = Alloc(X, Y, N, p)
%#codegen
%  추력 배분 — 요구 힘·모멘트를 세 추진기로 나눈다.
%
%    X = FL + FR                      전후력 [N]
%    Y = FB                           횡력 [N]  — 선수추진기만 낸다
%    N = (FL - FR)*b + l3*FB          요 모멘트 [N m]
%
%  p = [b; l3; Fmax; Fbmax]
%    b     half_beam   좌·우 추진기까지의 반폭 [m]
%    l3    l_bow       무게중심에서 선수추진기까지 [m]
%    Fmax  선미 추진기 추력 한계 [N],  Fbmax 선수추진기 추력 한계 [N]
%
%  선수추진기가 횡력을 내면 요 모멘트 l3*FB 가 딸려 온다. 그것을 좌·우
%  추진기가 되받아 빼야 선수각이 돌아가지 않는다 — 아래 N - l3*FB 가 그것이다.
b = p(1);  l3 = p(2);  Fmax = p(3);  Fbmax = p(4);
FB = Y;
if FB >  Fbmax, FB =  Fbmax; end
if FB < -Fbmax, FB = -Fbmax; end
%  포화된 뒤의 FB 로 모멘트를 센다 — 실제로 딸려 온 만큼만 되받는다
M  = N - l3*FB;
FL = X/2 + M/(2*b);
FR = X/2 - M/(2*b);
if FL >  Fmax, FL =  Fmax; end
if FL < -Fmax, FL = -Fmax; end
if FR >  Fmax, FR =  Fmax; end
if FR < -Fmax, FR = -Fmax; end

== matlab function W08_2_dock/Thrusters/F2n ==
  data: FL input; n_cmd output; FR input; FB input; k input; lim input
function n_cmd = F2n(FL, FR, FB, k, lim)
%#codegen
% Inverse propeller law:  F = k*n*|n|  ->  n = sign(F)*sqrt(|F|/k)
% lim 은 채널별 회전수 상한 — 선수추진기는 좌·우보다 작다
F = [FL; FR; FB];
n_cmd = zeros(3,1);
for i = 1:3
    ni = sign(F(i)) * sqrt(abs(F(i))/k);
    if ni >  lim(i), ni =  lim(i); end
    if ni < -lim(i), ni = -lim(i); end
    n_cmd(i) = ni;
end

== matlab function W08_2_dock/Thrusters/n2F ==
  data: n input; FL output; k input; FR output; FB output
function [FL, FR, FB] = n2F(n, k)
%#codegen
FL = k * n(1) * abs(n(1));
FR = k * n(2) * abs(n(2));
FB = k * n(3) * abs(n(3));

== matlab function W08_2_dock/MotionModel/EOM ==
  data: s input; xdot output; FL input; FR input; FB input; p input
function xdot = EOM(s, FL, FR, FB, p)
%#codegen
% 3-DOF WAM-V equations of motion, NED.
% Coefficients come straight from the Gazebo VRX plugins.
u = s(1); v = s(2); r = s(3); psi = s(6);
m=p(1); Izz=p(2); Xu=p(3); Xuu=p(4); Yv=p(5); Yvv=p(6);
Nr=p(7); Nrr=p(8); b_half=p(9); l3=p(10);

% 선수추진기는 **횡력**과 **요 모멘트**를 동시에 만든다 (l3 만큼 앞에 있다)
X = FL + FR;
Y = FB;
N = (FL - FR)*b_half + l3*FB;
Dx = (Xu + Xuu*abs(u))*u;
Dy = (Yv + Yvv*abs(v))*v;
Dn = (Nr + Nrr*abs(r))*r;

du = (X - Dx)/m + v*r;
dv = (Y - Dy)/m - u*r;
dr = (N - Dn)/Izz;

xdot = [du; dv; dr;
        u*cos(psi) - v*sin(psi);
        u*sin(psi) + v*cos(psi);
        r];

== matlab function W08_2_dock/MotionModel/States ==
  data: s input; x_n output; y_n output; psi output; u output; v output; r output; beta output
function [x_n, y_n, psi, u, v, r, beta] = States(s)
%#codegen
% v (횡속도) 를 하나 더 낸다 — 접안이 횡속도 고리로 돌아가므로
% 제어기도 화면도 v 를 읽는다. 실습 A~D 는 쓰지 않아 내보내지 않았다.
% chi (침로) 와 U (대지속력) 는 이 주차가 쓰지 않는다 (check_tags).
u = s(1); v = s(2); r = s(3);
x_n = s(4); y_n = s(5); psi = s(6);
beta = atan2(v, u);

== matlab function W08_2_dock/Animate/AnimateFcn ==
  data: x_n input; y_n input; psi input; mode input; turns input; psi_ref input; u input; ok output; gate_u input; FL input; FR input; idx input; phase input; v input; t input; en input
function ok = AnimateFcn(x_n, y_n, psi, mode, turns, psi_ref, u, gate_u, FL, FR, idx, phase, v, t, en)
%#codegen
% Live plot while the model runs. A MATLAB Function block cannot
% plot, so the drawing function is declared extrinsic: Simulink
% calls plain MATLAB instead of generating code for it.
coder.extrinsic('W08_dock_animate');
ok = 1;
if en > 0.5
    W08_dock_animate(x_n, y_n, psi, mode, turns, psi_ref, u, gate_u, FL, FR, idx, phase, v, t);
end

== matlab function W08_2_dock/Guidance/LoiterVF ==
  data: x_n input; psi_lo output; y_n input; x_c input; y_c input; rd input; pc input; r output; theta output
function [psi_lo, r, theta] = LoiterVF(x_n, y_n, x_c, y_c, rd, pc)
%#codegen
% Circular-orbit vector field guidance.
%   Jung, Lim, Lee, Bang, "Unmanned Aircraft Vector Field Path Following
%   with Arrival Angle Control".  eq. (9) + eq. (13), collapsed into the
%   single line the paper itself writes as eq. (30).
%
%   rd  desired orbit radius [m]
%   pc  shaping parameter.  SIGN sets the turn direction:
%         pc > 0  clockwise,   pc < 0  counter-clockwise
%       A smaller |pc| pulls the boat harder onto the circle.
%
% Speed does not appear here.  eq. (9) scales BOTH polar components by
% the same positive factor vd/sqrt((r-rd)^2+(pc*r)^2), and eq. (13)
% feeds them to atan2, which cannot see a positive common factor.  So
% the normalisation and vd cancel exactly and the course is just the
% bearing from the centre plus an angle off the radius line.  The boat
% gets its speed from u_cmd, not from the field.
%
% The crab angle is not subtracted here either, for the same reason as
% in week 7:  guidance names the course, control holds the heading.

dx = x_n - x_c;
dy = y_n - y_c;

r     = sqrt(dx*dx + dy*dy);      % distance from the centre
theta = atan2(dy, dx);            % bearing of the boat from the centre
if r < 1e-6, r = 1e-6; end        % the centre itself is singular

% eq. (30):  chi_d = theta + atan2(pc*r, -(r - rd))
%   r > rd  turn inward,   r < rd  turn outward,   r = rd  tangential
chi_d  = theta + atan2(pc*r, -(r - rd));
psi_lo = atan2(sin(chi_d), cos(chi_d));    % wrap to +-pi

== matlab function W08_2_dock/Guidance/WpManager ==
  data: x_n input; psi_los output; y_n input; wp_x input; wp_y input; Delta input; R input; loiter_wp input; mode input; idx_prev input; y_e output; idx output; at_loiter output; at_end output
function [psi_los, y_e, idx, at_loiter, at_end] = WpManager( ...
         x_n, y_n, wp_x, wp_y, Delta, R, loiter_wp, mode, idx_prev)
%#codegen
% Waypoint bookkeeping plus LOS guidance (week 7).
%   idx = index of the leg START. The leg runs wp(idx) -> wp(idx+1).
%   The index only advances while the mission is in waypoint mode,
%   so a loiter never makes the boat skip a leg.

n = numel(wp_x);
k = min(max(idx_prev, 1), n-1);

xk  = wp_x(k);    yk  = wp_y(k);
xk1 = wp_x(k+1);  yk1 = wp_y(k+1);

pi_p = atan2(yk1 - yk, xk1 - xk);
y_e  = -(x_n - xk)*sin(pi_p) + (y_n - yk)*cos(pi_p);
psi_los = pi_p - atan(y_e / Delta);

d_next  = sqrt((xk1 - x_n)^2 + (yk1 - y_n)^2);
reached = d_next <= R;

% arriving at the loiter waypoint, and arriving at the last one
if reached && ((k+1) == loiter_wp)
    at_loiter = 1;
else
    at_loiter = 0;
end
if reached && (k == n-1)
    at_end = 1;
else
    at_end = 0;
end

% advance only in waypoint mode
if (mode < 1.5) && reached && (k < n-1)
    idx = k + 1;
else
    idx = k;
end

== matlab function W08_2_dock/Guidance/TurnCount ==
  data: theta input; turns output; r input; rd input; mode input; th_prev input; acc_prev input; armed_prev input; th_out output; acc_out output; armed output
function [turns, th_out, acc_out, armed] = TurnCount( ...
         theta, r, rd, mode, th_prev, acc_prev, armed_prev)
%#codegen
% Count laps, but only while the mission is loitering (mode 2).
% Leaving loiter mode resets the counter, so a second loiter later
% starts from zero again.

th_out = theta;

if mode < 1.5 || mode > 2.5
    turns = 0; acc_out = 0; armed = 0;
    return
end

tol = 0.3*rd;
if armed_prev < 0.5
    acc_out = 0;
    if abs(r - rd) <= tol
        armed = 1;
    else
        armed = 0;
    end
else
    armed = 1;
    d = theta - th_prev;
    d = atan2(sin(d), cos(d));
    acc_out = acc_prev + d;
end
turns = abs(acc_out) / (2*pi);

== matlab function W08_2_dock/Guidance/BerthRef ==
  data: x_n input; y_n input; psi input; u input; x_ref output; mode input; q input; ph_prev input; y_ref output; psi_dock output; gate_d output; phase output
function [x_ref, y_ref, psi_dock, gate_d, phase] = BerthRef( ...
         x_n, y_n, psi, u, mode, q, ph_prev)
%#codegen
% 접안 기준점 — 위치제어(OuterLoop)가 따라갈 점 하나와 선수각 하나를 낸다.
%
%   q = [dx; dy; dpsi; La; sd; Rd; Rs]
%     dx,dy  접안 완료점(베이 안) [m, NED]
%     dpsi   접안 자세 — 부두와 나란한 선수각 [rad]
%     La     접근점까지의 거리 [m],  sd 접안하는 쪽 (+1 우현 / -1 좌현)
%     Rd     접근점 도착 반경 [m],   Rs 접안 완료 반경 [m]
%
%   단계 phase
%     0  접근점으로 — 선수각은 접근점을 바라본다
%     1  선수각 맞추기 — 접근점에 묶어 두고 부두와 나란해지며 멈출 때까지
%     2  순수 옆걸음 — 기준점만 베이 안으로 옮긴다. 선수각은 그대로
%     3  접안 완료 — 기준점을 선석에 두고 위치제어로 자리를 지킨다
dx = q(1);  dy = q(2);  dpsi = q(3);  La = q(4);
sd = q(5);  Rd = q(6);  Rs   = q(7);

%  접근점 — 접안점에서 부두 바깥으로 La 만큼 떨어진 점
ax = dx - sd*La*sin(dpsi);
ay = dy + sd*La*cos(dpsi);

ph = ph_prev;
if mode < 2.5
    %  아직 도킹 차례가 아니다. 단계를 0 으로 되돌리고 기준점은 제자리에 둔다
    %  (위치 오차 0 — OuterLoop 이 돌고 있어도 지령을 내지 않는다)
    ph = 0;  x_ref = x_n;  y_ref = y_n;  psi_dock = dpsi;
elseif ph < 0.5
    x_ref = ax;  y_ref = ay;  psi_dock = atan2(ay - y_n, ax - x_n);
    if sqrt((ax - x_n)^2 + (ay - y_n)^2) < Rd, ph = 1; end
elseif ph < 1.5
    x_ref = ax;  y_ref = ay;  psi_dock = dpsi;
    e = atan2(sin(dpsi - psi), cos(dpsi - psi));
    %  옆걸음은 **배가 멈춘 뒤** 시작한다. 전후 속력이 남아 있으면
    %  앞으로 미끄러지며 옆으로 가 궤적이 비스듬해진다 — 순수 옆걸음이 아니다
    if abs(e) < 5*pi/180 && abs(u) < 0.20, ph = 2; end
else
    x_ref = dx;  y_ref = dy;  psi_dock = dpsi;
    if sqrt((dx - x_n)^2 + (dy - y_n)^2) < Rs, ph = 3; end
end

phase  = ph;

%  gate_d — 위치제어 문. 접안 차례가 되면 열고 **접안 뒤에도 닫지 않는다**.
%  2026-11-01 측정에서 드러난 것 — ph = 3 에서 문을 닫으면 횡 PI 적분기가
%  마지막 값(약 96 N)에 얼어붙은 채 남아 선수추진기가 계속 밀고, 배는 선석을
%  지나 베이 뒤 벽을 뚫는다 (10 s 에 6.0 m). **오차를 끊는 문은 적분기를 0 으로
%  되돌리지 않는다.** 멈추려면 오차를 끊지 말고 받아야 한다 — 선석에 가까워질수록
%  위치 오차가 줄어 횡 속도 지령이 스스로 0 이 되고, 그것이 제동이다
gate_d = double(mode > 2.5);

== stateflow chart W08_2_dock/Mission/MissionFSM ==
  settings: updateMethod=DISCRETE  sampleTime=Ts_ctrl
  state WpFollow
    en: mode = 1;
  state Dock
    en: mode = 3;
  state Finish
    en: mode = 4;
  state Loiter
    en: mode = 2;
  (default) -> WpFollow
  Loiter -> WpFollow : [turns >= req_turns]
  WpFollow -> Dock [order 2] : [at_end > 0.5]
  Dock -> Finish : [phase > 2.5]
  WpFollow -> Loiter [order 1] : [at_loiter > 0.5]
  data: at_loiter input; turns input; req_turns input; at_end input; phase input; mode output
